simulink model "Circuito_Online_Definitivo"  (R2024b)
settings: Solver=FixedStepAuto  StartTime=0.0  StopTime=60  RelTol=1e-3
model workspace (MAT data in the model file):
  PCA_coeffK : Simulink.Parameter (value not decoded)
  PCA_mu : Simulink.Parameter (value not decoded)
  PCA_sigma : Simulink.Parameter (value not decoded)
  coeffK29 = [0.031417995941 -0.0136921286523 0.101212984636 0.106176563865 0.0788268242014 -0.0826314602301 0.096815718661 0.100927555615 0.105773936814 0.00647840331643 0.0950185241378 0.0183038808121 ... (4698 elements, 162x29)]
  k_optimum = 43
  k_optimum29 = 29
  mu29 = [0.0561230714509 -0.282261972362 6.94500497276 2.31958575633 8.7597365107 -8.35900443597 17.1187409467 5440.0049078 2.35464218965 4.55157780819 701.708188274 0.88671875 ... (162 elements, 1x162)]
  sigma29 = [0.34168385245 0.471736845585 6.86251142603 1.25143636865 6.83836988941 5.25913074711 10.0563900959 5299.20213776 1.23002081301 1.39530906556 587.851063427 0.97569014465 ... (162 elements, 1x162)]
symbols that are objects in the model workspace (value not decoded): PCA_coeffK, PCA_mu, PCA_sigma
libraries: visionsources x3, androidsensorlib x2, androiduilib x1, androidaudiovideolib x1
(part 2 of 2)

== matlab function Circuito_Online_Definitivo/Finestratura1 ==
  data: acc_x input; acc_x_win output; acc_y input; acc_z input; gyro_x input; gyro_y input; gyro_z input; acc_y_win output; acc_z_win output; gyr_x_win output; gyr_y_win output; gyr_z_win output; window6 output; valid output
function [acc_x_win, acc_y_win, acc_z_win, ...
          gyr_x_win, gyr_y_win, gyr_z_win, window6, valid] = ...
          Finestratura_RAW(acc_x, acc_y, acc_z, gyro_x, gyro_y, gyro_z)
%#codegen
% Finestratura online su segnali GREZZI (primo step della pipeline)
% In: campioni live (sample-by-sample)
% Out: finestra completa (winLen x 1) + window6 (6 x winLen) + valid (pulse)

% ====== PARAMETRI (coerenti col training) ======
preSamples   = int32(200);
postSamples  = int32(569);     % totale winLen = 200 + 1 + 569 = 770
threshold    = single(1.7);
refractoryN  = int32(100);     % anti doppio trigger (campioni)

winLen = int32(preSamples + 1 + postSamples);

% ====== PERSISTENT ======
persistent preBufAx preBufAy preBufAz preBufGx preBufGy preBufGz
persistent preIdx
persistent state postCount
persistent winAx winAy winAz winGx winGy winGz
persistent refractoryCount

if isempty(state)
    % pre-trigger ring buffer (ultimi preSamples campioni)
    preBufAx = zeros(preSamples,1,'single');
    preBufAy = zeros(preSamples,1,'single');
    preBufAz = zeros(preSamples,1,'single');
    preBufGx = zeros(preSamples,1,'single');
    preBufGy = zeros(preSamples,1,'single');
    preBufGz = zeros(preSamples,1,'single');
    preIdx   = int32(1);

    % state: 0=idle, 1=collect post
    state = int32(0);
    postCount = int32(0);

    % finestra completa
    winAx = zeros(winLen,1,'single');
    winAy = zeros(winLen,1,'single');
    winAz = zeros(winLen,1,'single');
    winGx = zeros(winLen,1,'single');
    winGy = zeros(winLen,1,'single');
    winGz = zeros(winLen,1,'single');

    refractoryCount = int32(0);
end

% ====== CAST ingressi a single ======
acc_x  = single(acc_x);  acc_y  = single(acc_y);  acc_z  = single(acc_z);
gyro_x = single(gyro_x); gyro_y = single(gyro_y); gyro_z = single(gyro_z);

% ====== OUTPUT di default (dimensioni fisse) ======
acc_x_win = zeros(winLen,1,'single');
acc_y_win = zeros(winLen,1,'single');
acc_z_win = zeros(winLen,1,'single');
gyr_x_win = zeros(winLen,1,'single');
gyr_y_win = zeros(winLen,1,'single');
gyr_z_win = zeros(winLen,1,'single');
window6   = zeros(6, winLen,'single');
valid     = false;

% ====== aggiorna sempre il pre-buffer circolare ======
preBufAx(preIdx) = acc_x;
preBufAy(preIdx) = acc_y;
preBufAz(preIdx) = acc_z;
preBufGx(preIdx) = gyro_x;
preBufGy(preIdx) = gyro_y;
preBufGz(preIdx) = gyro_z;

preIdx = preIdx + 1;
if preIdx > preSamples
    preIdx = int32(1);
end

% ====== decrementa refractory ======
if refractoryCount > 0
    refractoryCount = refractoryCount - 1;
end

% ====== trigger per segmentazione (qui: acc_x grezzo) ======
triggerSignal = acc_x;

% ====== macchina a stati ======
if state == 0
    % IDLE: aspetta trigger
    if (refractoryCount == 0) && (triggerSignal > threshold)

        % ---- copia gli ultimi preSamples campioni in ordine temporale ----
        % preIdx punta alla prossima cella da scrivere -> il più vecchio è preIdx
        k = int32(1);
        for n = int32(0):(preSamples-1)
            idx = preIdx + n;
            if idx > preSamples
                idx = idx - preSamples;
            end
            winAx(k) = preBufAx(idx);
            winAy(k) = preBufAy(idx);
            winAz(k) = preBufAz(idx);
            winGx(k) = preBufGx(idx);
            winGy(k) = preBufGy(idx);
            winGz(k) = preBufGz(idx);
            k = k + 1;
        end

        % ---- campione di trigger (corrente) come elemento preSamples+1 ----
        winAx(preSamples+1) = acc_x;
        winAy(preSamples+1) = acc_y;
        winAz(preSamples+1) = acc_z;
        winGx(preSamples+1) = gyro_x;
        winGy(preSamples+1) = gyro_y;
        winGz(preSamples+1) = gyro_z;

        % passa allo stato di raccolta post
        postCount = int32(0);
        state = int32(1);

        % anti doppio trigger
        refractoryCount = refractoryN;
    end

else
    % COLLECT POST: riempi elementi (preSamples+2) .. winLen
    postCount = postCount + 1;
    pos = preSamples + 1 + postCount;

    winAx(pos) = acc_x;
    winAy(pos) = acc_y;
    winAz(pos) = acc_z;
    winGx(pos) = gyro_x;
    winGy(pos) = gyro_y;
    winGz(pos) = gyro_z;

    if postCount >= postSamples
        % finestra completa pronta: emetti per 1 step
        acc_x_win = winAx;
        acc_y_win = winAy;
        acc_z_win = winAz;
        gyr_x_win = winGx;
        gyr_y_win = winGy;
        gyr_z_win = winGz;

        window6 = [winAx.'; winAy.'; winAz.'; winGx.'; winGy.'; winGz.']; % 6 x winLen
        valid = true;

        % ritorna in idle
        state = int32(0);
    end
end
end

== matlab function Circuito_Online_Definitivo/Filter1 ==
  data: window6 input; window6_filt output; valid input; outValid output
function [window6_filt, outValid] = FilterWindow_filtfilt(window6, valid)
%#codegen
% Filtraggio zero-phase (filtfilt) su finestra completa (6 x winLen)
% In:  window6 (6 x winLen), valid (bool)
% Out: window6_filt (6 x winLen), outValid (bool)

% ==== PARAMETRI FILTRO ====
fs          = 200;
low_cutoff  = 0.021;
high_cutoff = 25;
n           = 2;

% ==== LUNGHEZZA FINESTRA (fissa) ====
winLen = 770;   % <-- cambia qui se la tua finestra non è 770

% ==== COEFFICIENTI PERSISTENTI ====
persistent b a
if isempty(b)
    [b_d, a_d] = butter(n, [low_cutoff high_cutoff]/(fs/2), 'bandpass');
    % filtfilt lavora meglio in double: teniamo i coeff in double
    b = b_d;
    a = a_d;
end

% ==== OUTPUT DEFAULT ====
window6_filt = zeros(6, winLen, 'single');
outValid = false;

% ==== ESEGUI SOLO QUANDO LA FINESTRA È PRONTA ====
if valid
    outValid = true;

    % Filtra ciascun canale (righe: 1..6)
    for ch = 1:6
        x = double(window6(ch, :)).';      % colonna winLen x 1
        y = filtfilt(b, a, x);             % zero-phase
        window6_filt(ch, :) = single(y).'; % torna a riga
    end
end

end

== matlab function Circuito_Online_Definitivo/Finestratura ==
  data: filtered_acc_x input; acc_x_finestrato output; filtered_acc_y input; filtered_acc_z input; filtered_gyro_x input; filtered_gyro_y input; filtered_gyro_z input; acc_y_finestrato output; acc_z_finestrato output; gyr_x_finestrato output; gyr_y_finestrato output; gyr_z_finestrato output; window6 output; valid output
function [acc_x_finestrato, acc_y_finestrato, acc_z_finestrato, ...
          gyr_x_finestrato, gyr_y_finestrato, gyr_z_finestrato, window6, valid] = ...
          Finestratura( filtered_acc_x, filtered_acc_y, filtered_acc_z, ...
                        filtered_gyro_x, filtered_gyro_y, filtered_gyro_z )
%#codegen

% ====== PARAMETRI (devono combaciare col training) ======
preSamples  = 200;
postSamples = 569;      % 200 + 1 + 499 = 700 campioni totali
threshold   = 1.7;

winLen = preSamples + 1 + postSamples;

% ====== PERSISTENT: memoria tra step ======
persistent preBufAx preBufAy preBufAz preBufGx preBufGy preBufGz
persistent preIdx
persistent state postCount
persistent winAx winAy winAz winGx winGy winGz
persistent refractoryCount

if isempty(state)
    % buffer circolare pre-trigger (ultimi 200 campioni)
    preBufAx = zeros(preSamples,1);
    preBufAy = zeros(preSamples,1);
    preBufAz = zeros(preSamples,1);
    preBufGx = zeros(preSamples,1);
    preBufGy = zeros(preSamples,1);
    preBufGz = zeros(preSamples,1);
    preIdx   = 1;

    % state: 0=idle, 1=collect post
    state = int32(0);
    postCount = int32(0);

    % finestra completa (700) pronta quando finita
    winAx = zeros(winLen,1);
    winAy = zeros(winLen,1);
    winAz = zeros(winLen,1);
    winGx = zeros(winLen,1);
    winGy = zeros(winLen,1);
    winGz = zeros(winLen,1);

    % anti doppio-trigger (in campioni)
    refractoryCount = int32(0);
end

% ====== OUTPUT di default ======
acc_x_finestrato = zeros(winLen,1);
acc_y_finestrato = zeros(winLen,1);
acc_z_finestrato = zeros(winLen,1);
gyr_x_finestrato = zeros(winLen,1);
gyr_y_finestrato = zeros(winLen,1);
gyr_z_finestrato = zeros(winLen,1);
valid = false;
window6 = zeros(6,winLen);

% ====== aggiorna sempre il pre-buffer circolare ======
preBufAx(preIdx) = filtered_acc_x;
preBufAy(preIdx) = filtered_acc_y;
preBufAz(preIdx) = filtered_acc_z;
preBufGx(preIdx) = filtered_gyro_x;
preBufGy(preIdx) = filtered_gyro_y;
preBufGz(preIdx) = filtered_gyro_z;

preIdx = preIdx + 1;
if preIdx > preSamples
    preIdx = 1;
end

% ====== decrementa refractory ======
if refractoryCount > 0
    refractoryCount = refractoryCount - 1;
end

% ====== trigger usato per la segmentazione (qui: acc_x filtrato) ======
triggerSignal = filtered_acc_x;

% ====== macchina a stati ======
if state == 0
    % IDLE: aspetta trigger
    if (refractoryCount == 0) && (triggerSignal > threshold)

        % ---- copia gli ultimi 200 campioni in ordine temporale ----
        % preIdx punta alla prossima cella da scrivere -> il più vecchio è preIdx
        k = int32(1);
        for n = 0:(preSamples-1)
            idx = preIdx + n;
            if idx > preSamples
                idx = idx - preSamples;
            end
            winAx(k) = preBufAx(idx);
            winAy(k) = preBufAy(idx);
            winAz(k) = preBufAz(idx);
            winGx(k) = preBufGx(idx);
            winGy(k) = preBufGy(idx);
            winGz(k) = preBufGz(idx);
            k = k + 1;
        end

        % ---- campione di trigger (quello corrente) come elemento 201 ----
        winAx(preSamples+1) = filtered_acc_x;
        winAy(preSamples+1) = filtered_acc_y;
        winAz(preSamples+1) = filtered_acc_z;
        winGx(preSamples+1) = filtered_gyro_x;
        winGy(preSamples+1) = filtered_gyro_y;
        winGz(preSamples+1) = filtered_gyro_z;

        % passa allo stato di raccolta post
        postCount = int32(0);
        state = int32(1);

        % anti doppio trigger (~0.5s a 200Hz = 100 campioni)
        refractoryCount = int32(100);
    end

else
    % COLLECT POST: riempi elementi 202..700
    postCount = postCount + 1;
    pos = preSamples + 1 + postCount;

    winAx(pos) = filtered_acc_x;
    winAy(pos) = filtered_acc_y;
    winAz(pos) = filtered_acc_z;
    winGx(pos) = filtered_gyro_x;
    winGy(pos) = filtered_gyro_y;
    winGz(pos) = filtered_gyro_z;

    if postCount >= postSamples
        % finestra completa pronta: emetti per 1 step
        acc_x_finestrato = winAx;
        acc_y_finestrato = winAy;
        acc_z_finestrato = winAz;
        gyr_x_finestrato = winGx;
        gyr_y_finestrato = winGy;
        gyr_z_finestrato = winGz;
        valid = true;
        window6 = [winAx.'; winAy.'; winAz.'; winGx.'; winGy.'; winGz.'];  % 6 x winLen

        % ritorna in idle
        state = int32(0);


    end
end
end

== matlab function Circuito_Online_Definitivo/Filter ==
  data: acc_x input; filtered_acc_x output; acc_y input; acc_z input; gyro_x input; gyro_y input; gyro_z input; filtered_acc_y output; filtered_acc_z output; filtered_gyro_x output; filtered_gyro_y output; filtered_gyro_z output
function [filtered_acc_x, filtered_acc_y, filtered_acc_z, ...
          filtered_gyro_x, filtered_gyro_y, filtered_gyro_z] = fcn(acc_x, acc_y, acc_z, gyro_x, gyro_y, gyro_z)
%#codegen

    % Parametri
    fs = single(200);
    low_cutoff  = single(0.021);
    high_cutoff = single(25);
    n = 2;

    persistent b a zax zay zaz zgx zgy zgz nst
    if isempty(b)
        [b_d,a_d] = butter(n, double([low_cutoff high_cutoff])/(double(fs)/2), 'bandpass');
        b = single(b_d);
        a = single(a_d);

        nst = int32(max(length(a), length(b)) - 1);

        zax = zeros(nst,1,'single'); zay = zeros(nst,1,'single'); zaz = zeros(nst,1,'single');
        zgx = zeros(nst,1,'single'); zgy = zeros(nst,1,'single'); zgz = zeros(nst,1,'single');
    end

    % Cast ingressi a single (se già single, non cambia)
    acc_x  = single(acc_x);  acc_y  = single(acc_y);  acc_z  = single(acc_z);
    gyro_x = single(gyro_x); gyro_y = single(gyro_y); gyro_z = single(gyro_z);

    % Filtraggio sample-by-sample
    [filtered_acc_x, zax]  = filter(b, a, acc_x,  zax);
    [filtered_acc_y, zay]  = filter(b, a, acc_y,  zay);
    [filtered_acc_z, zaz]  = filter(b, a, acc_z,  zaz);

    [filtered_gyro_x, zgx] = filter(b, a, gyro_x, zgx);
    [filtered_gyro_y, zgy] = filter(b, a, gyro_y, zgy);
    [filtered_gyro_z, zgz] = filter(b, a, gyro_z, zgz);
end

== matlab function Circuito_Online_Definitivo/Feature Extraciton ==
  data: window6_filt input; features_out output; outValid output; valid input
function [features_out, outValid] = feature_extraction_online(window6_filt, valid)
%FEATURE_EXTRACTION_ONLINE  Online (1 finestra -> 1 vettore feature)
% Input:
%   window6 : 6x770  (assi x campioni)
%   valid   : boolean (true quando finestra completa)
% Output:
%   features_out : 1x162 double (feature concatenate)
%   outValid     : copia di valid
%
%#codegen

outValid = valid;

% Dimensione feature
F = 162;

% Preallocazione (codegen-friendly, dimensione fissa)
features_out = zeros(1, F);

if ~valid
    return;
end

% Parametri (come offline)
Fs = 200;
N_win = 256;

% Porta nel formato N x 6 (campioni x assi)
signals = window6_filt.';   % 770x6

% Indice di scrittura nel vettore finale
k = 1;

% ===== Feature per asse (6 canali) =====
for ch = 1:6
    sig = signals(:, ch);

    ft  = funzione_dominio_tempo(sig);                  % 1x10
    ff  = funzione_dominio_frequenza(sig, Fs, N_win);   % 1x8
    fTF = funzione_dominio_tempofrequenza(sig, Fs, N_win); % 1x6 (senza wavelet)

    % Forza riga (sicurezza)
    ft  = ft(:).';
    ff  = ff(:).';
    fTF = fTF(:).';

    % Copia nel vettore finale
    n = numel(ft);  features_out(1, k:k+n-1) = ft;  k = k + n;
    n = numel(ff);  features_out(1, k:k+n-1) = ff;  k = k + n;
    n = numel(fTF); features_out(1, k:k+n-1) = fTF; k = k + n;
end

% ===== Feature multi-asse (acc + gyro) =====
f_acc  = funzione_multiasse(signals(:,1:3));   % 1x9
f_gyro = funzione_multiasse(signals(:,4:6));   % 1x9

f_acc  = f_acc(:).';
f_gyro = f_gyro(:).';

n = numel(f_acc);  features_out(1, k:k+n-1) = f_acc;  k = k + n;
n = numel(f_gyro); features_out(1, k:k+n-1) = f_gyro; k = k + n;

end

== matlab function Circuito_Online_Definitivo/Hold_label ==
  data: label_in input; label_stable output; valid input
function label_stable = HoldLabel(label_in, valid) %#codegen
% label_in: int32  (uscita ML: -1 fermo, 1 passo1, 2 passo2)
% valid   : boolean (true SOLO quando finestra pronta)
% label_stable: int32 (label mantenuta, con ritorno automatico a fermo)

% === PARAMETRI ===
Fs = 200;                      % Hz (tuo sample rate)
timeout_sec = 2;             % dopo quanti secondi senza valid => FERMO
timeout_samples = int32(Fs * timeout_sec);

FERMO_LABEL = int32(-1);

persistent lastLabel noValidCount

if isempty(lastLabel)
    lastLabel = FERMO_LABEL;      % inizializza a fermo
    noValidCount = int32(0);
end

if valid
    % nuova decisione valida
    lastLabel = label_in;
    noValidCount = int32(0);
else
    % nessuna finestra valida: conta i campioni
    if noValidCount < timeout_samples
        noValidCount = noValidCount + int32(1);
    end

    % se passa troppo tempo senza eventi, torna a fermo
    if noValidCount >= timeout_samples
        lastLabel = FERMO_LABEL;
    end
end

label_stable = lastLabel;
end

== matlab function Circuito_Online_Definitivo/PCA ==
  data: x_raw input; x_pca output double size=[1 43]; xPcaValid output; valid input; PCA_mu input; PCA_sigma input; PCA_coeffK input
% function [x_pca, xPcaValid] = ApplyPCA(x_raw, valid)
% %#codegen
% 
% xPcaValid = valid;
% 
% persistent mu sigma coeffK k
% if isempty(mu)
%     S = load('pca_params.mat','mu','sigma','coeffK','k_optimum');
%     mu = double(S.mu);
%     sigma = double(S.sigma);
%     coeffK = double(S.coeffK);
%     k = int32(S.k_optimum);
% end
% 
% x_pca = zeros(1, double(k), 'double');
% 
% if ~valid
%     return;
% end
% 
% x_std = (x_raw - mu) ./ (sigma + eps);
% x_pca = x_std * coeffK;
% 
% end

function [x_pca, xPcaValid] = ApplyPCA(x_raw, valid, PCA_mu, PCA_sigma, PCA_coeffK) %#codegen
%function [x_pca, xPcaValid] = ApplyPCA(x_raw, valid, mu29, sigma29, coeffK29) %#codegen
xPcaValid = valid;

x_pca = zeros(1, 43, 'double');
%x_pca = zeros(1, 29, 'double');

if ~valid
    return;
end

% Forza riga 1x162 (fondamentale)
x   = double(x_raw(:)).';       % 1x162
mu  = double(PCA_mu(:)).';      % 1x162
sig = double(PCA_sigma(:)).';   % 1x162
C   = double(PCA_coeffK);       % 162x43
% x   = double(x_raw(:)).';       % 1x162
% mu  = double(mu29(:)).';      % 1x162
% sig = double(sigma29(:)).';   % 1x162
% C   = double(coeffK29);       % 162x43

x_std = (x - mu) ./ (sig + eps);   % 1x162
x_pca = x_std * C;                 % 1x43

end

== matlab function Circuito_Online_Definitivo/ML ==
  data: x_pca input; label output; valid input
function label = fcn(x_pca, valid) %#codegen
% x_pca : 1x43 double
% valid : boolean
% label : int32 (classe predetta, -1 se non valida)

persistent mdl

% Carica il modello UNA SOLA VOLTA
if isempty(mdl)
    mdl = loadLearnerForCoder("best_svm_model_onlyFILT.mat");
    %mdl = loadLearnerForCoder("ML_albero_ottimizzata.mat");
end

% Preallocazione FISSA del tipo (fondamentale)
label = int32(-1);

% Se la finestra non è valida, esci
if ~valid
    return;
end

% Predizione (ritorna double)
y = predict(mdl, x_pca);

% Cast esplicito a int32 (codegen-safe)
label = int32(y);

end

== matlab function Circuito_Online_Definitivo/LabelToImmage ==
  data: label_stable input; img_idx output
function img_idx = LabelToImageIndex(label_stable) %#codegen
% label_stable: int32 (-1 fermo, 1 passo1, 2 passo2)
% img_idx: uint8 (1=passo1, 2=passo2, 3=fermo)

% default: fermo
img_idx = uint8(3);

if label_stable == int32(1)
    img_idx = uint8(1);
elseif label_stable == int32(2)
    img_idx = uint8(2);
elseif label_stable == int32(-1)
    img_idx = uint8(3);
end
end

== matlab function Circuito_Online_Definitivo/SplitRGB ==
  data: img input; R output; G output; B output
function [R,G,B] = SplitRGB(img) %#codegen
% img: uint8 [H x W x C] dove C può essere 1 o 3
% R,G,B: uint8 [H x W]

% Prendo H e W in modo codegen-safe
H = size(img,1);
W = size(img,2);

% Prealloc
R = zeros(H, W, 'like', img);
G = zeros(H, W, 'like', img);
B = zeros(H, W, 'like', img);

% Se RGB vero
if ndims(img) == 3 && size(img,3) == 3
    R = img(:,:,1);
    G = img(:,:,2);
    B = img(:,:,3);
else
    % Se è 1 canale (grayscale), lo replico
    R = img(:,:,1);
    G = img(:,:,1);
    B = img(:,:,1);
end
end
